simulink model "ex2"  (R2025b)
settings: Solver=VariableStepAuto  StartTime=0.0  StopTime=0.6  FixedStep=1e-4  RelTol=1e-4
values from neighbouring files (symbols this model uses):
  al = ap * 10    [sim3.m]
  Id_ref = psi_nominal_pu*psi_base/L_M    [sim3.m]
  Iq_ref = Te_nominal / ((3/2*K^2) * np * psi_nominal_pu*psi_base)    [sim3.m]
  ki = ac*(R_s+R_R+R_a)    [sim3.m]
  kip = ap*ap/psi_nominal    [sim3.m]
  kp = ac*L_sig    [sim3.m]
  kpp = 2*ap/psi_nominal    [sim3.m]
  L_sig = 0.0416    [sim3.m]
  R_a = ac*L_sig -(R_s+R_R)    [sim3.m]
  Te_nominal = Te_base * k    [sim3.m]
settings Model: Creator=Dimitris  LastModifiedBy=Dimitris

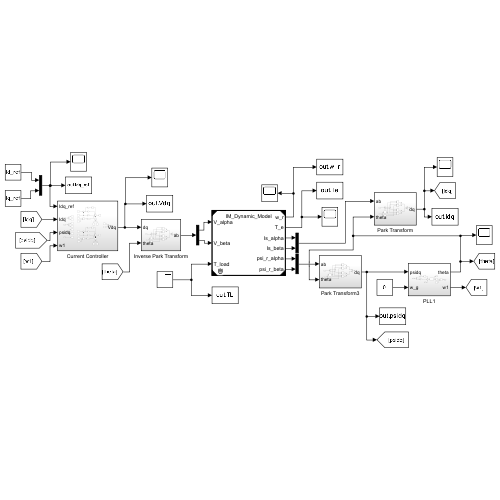
[thumbnail: Simulink's stored preview of the top-level diagram]
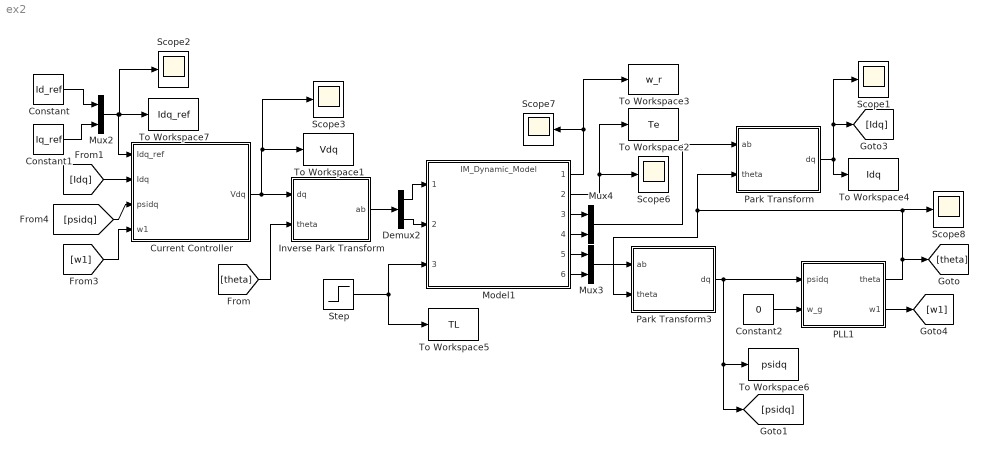
== system ex2 ==
  Constant : Constant  Value=Id_ref
  Constant1 : Constant  Value=Iq_ref
  Constant2 : Constant  Value=0
  Current Controller : Subsystem
  Demux2 : Demux  Outputs=2
  Inverse Park Transform : Subsystem
  Model1 : ModelReference  ModelNameDialog=IM_Dynamic_Model.slxp  ModelReferenceVersion=1.0  CopyOfModelProtected=on
  Mux2 : Mux  Inputs=2
  Mux3 : Mux  Inputs=2
  Mux4 : Mux  Inputs=2
  PLL1 : Subsystem
  Park Transform : Subsystem
  Park Transform3 : Subsystem
  Scope{1..3,6..8} (6 alike) : Scope
      Scope1 settings: ActiveDisplayYMinimum=-1.5675361173951203  ActiveDisplayYMaximum=7.0785524882099722
      Scope2 settings: ActiveDisplayYMinimum=0.8  ActiveDisplayYMaximum=2.8  DataLoggingVariableName=ScopeData2
      Scope3 settings: ActiveDisplayYMinimum=-366.50801253173779  ActiveDisplayYMaximum=2052.3481135758693  DataLoggingVariableName=ScopeData3
      Scope6 settings: ActiveDisplayYMinimum=-2.2517619671531257  ActiveDisplayYMaximum=20.265857704375257
      Scope7 settings: ActiveDisplayYMinimum=-65.744428661718672  ActiveDisplayYMaximum=591.69985795532909  DataLoggingVariableName=ScopeData6
      Scope8 settings: ActiveDisplayYMinimum=-0.78539816339744806  ActiveDisplayYMaximum=7.0685834705770345  DataLoggingVariableName=ScopeData7
  Step : Step  Time=0.3  After=Te_nominal*0.8  SampleTime=0
  To Workspace1 : ToWorkspace  VariableName=Vdq  SaveFormat=Timeseries  SampleTime=-1
  To Workspace2 : ToWorkspace  VariableName=Te  SaveFormat=Timeseries  SampleTime=-1
  To Workspace3 : ToWorkspace  VariableName=w_r  SaveFormat=Timeseries  SampleTime=-1
  To Workspace4 : ToWorkspace  VariableName=Idq  SaveFormat=Timeseries  SampleTime=-1
  To Workspace5 : ToWorkspace  VariableName=TL  SaveFormat=Timeseries  SampleTime=-1
  To Workspace6 : ToWorkspace  VariableName=psidq  SaveFormat=Timeseries  SampleTime=-1
  To Workspace7 : ToWorkspace  VariableName=Idq_ref  SaveFormat=Timeseries  SampleTime=-1
  wires:
  Current Controller/1(Vdq) -> Scope3/1, To Workspace1/1, Inverse Park Transform/1(dq)
  [Idq] -> Current Controller/2(Idq)
  Mux2/1 -> Scope2/1, To Workspace7/1, Current Controller/1(Idq_ref)
  Constant1/1 -> Mux2/2
  Constant/1 -> Mux2/1
  Inverse Park Transform/1(ab) -> Demux2/1
  PLL1/1(theta) -> Scope8/1, Park Transform3/2(theta), Park Transform/2(theta), [theta]
  Constant2/1 -> PLL1/2(w_g)
  Model1/4 -> Mux4/2
  Mux4/1 -> Park Transform/1(ab)
  Demux2/1 -> Model1/1
  Park Transform/1(dq) -> To Workspace4/1, [Idq], Scope1/1
  Step/1 -> To Workspace5/1, Model1/3
  Mux3/1 -> Park Transform3/1(ab)
  Demux2/2 -> Model1/2
  Model1/3 -> Mux4/1
  Model1/2 -> To Workspace2/1, Scope6/1
  Model1/6 -> Mux3/2
  Park Transform3/1(dq) -> [psidq], To Workspace6/1, PLL1/1(psidq)
  Model1/1 -> To Workspace3/1, Scope7/1
  Model1/5 -> Mux3/1
  [theta] -> Inverse Park Transform/2(theta)
  [psidq] -> Current Controller/3(psidq)
  [w1] -> Current Controller/4(w1)
  PLL1/2(w1) -> [w1]

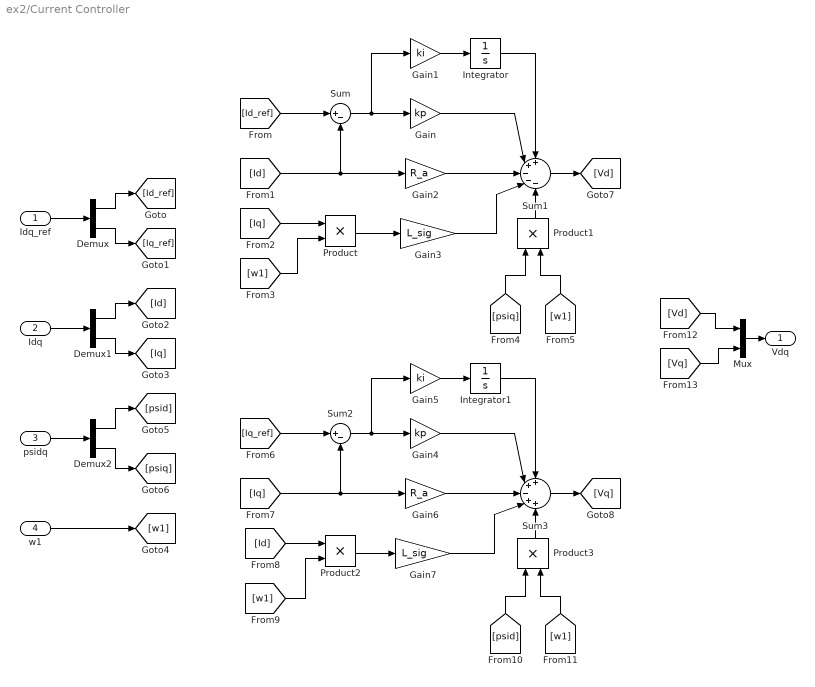
== system ex2/Current Controller ==
  Idq_ref : Inport
  Idq : Inport  Port=2
  psidq : Inport  Port=3
  w1 : Inport  Port=4
  Demux : Demux  Outputs=2
  Demux1 : Demux  Outputs=2
  Demux2 : Demux  Outputs=2
  Gain : Gain  Gain=kp
  Gain1 : Gain  Gain=ki
  Gain2 : Gain  Gain=R_a
  Gain3 : Gain  Gain=L_sig
  Gain4 : Gain  Gain=kp
  Gain5 : Gain  Gain=ki
  Gain6 : Gain  Gain=R_a
  Gain7 : Gain  Gain=L_sig
  Integrator : Integrator
  Integrator1 : Integrator
  Mux : Mux  Inputs=2
  Product{,1..3} (4 alike) : Product
  Sum : Sum  Inputs=|+-
  Sum1 : Sum  Inputs=++---
  Sum2 : Sum  Inputs=|+-
  Sum3 : Sum  Inputs=++-++
  Vdq : Outport
  wires:
  Idq_ref/1 -> Demux/1
  Mux/1 -> Vdq/1
  Idq/1 -> Demux1/1
  Demux/1 -> [Id_ref]
  Demux/2 -> [Iq_ref]
  Demux1/1 -> [Id]
  Demux1/2 -> [Iq]
  [Id_ref] -> Sum/1
  [Id] -> Sum/2, Gain2/1
  Sum/1 -> Gain1/1, Gain/1
  Gain1/1 -> Integrator/1
  Integrator/1 -> Sum1/1
  Gain/1 -> Sum1/2
  Gain2/1 -> Sum1/3
  Gain3/1 -> Sum1/4
  Product/1 -> Gain3/1
  w1/1 -> [w1]
  [Iq] -> Product/1
  [w1] -> Product/2
  psidq/1 -> Demux2/1
  Demux2/1 -> [psid]
  Demux2/2 -> [psiq]
  [psiq] -> Product1/1
  [w1] -> Product1/2
  Product1/1 -> Sum1/5
  Product3/1 -> Sum3/5
  [w1] -> Product3/2
  [psid] -> Product3/1
  Product2/1 -> Gain7/1
  [Id] -> Product2/1
  Integrator1/1 -> Sum3/1
  Gain6/1 -> Sum3/3
  Gain5/1 -> Integrator1/1
  Gain7/1 -> Sum3/4
  Sum2/1 -> Gain5/1, Gain4/1
  [Iq_ref] -> Sum2/1
  [w1] -> Product2/2
  [Iq] -> Sum2/2, Gain6/1
  Gain4/1 -> Sum3/2
  Sum1/1 -> [Vd]
  [Vd] -> Mux/1
  Sum3/1 -> [Vq]
  [Vq] -> Mux/2

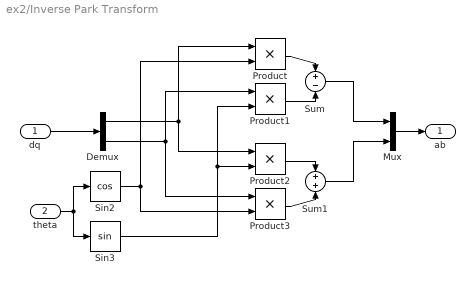
== system ex2/Inverse Park Transform ==
  dq : Inport
  theta : Inport  Port=2
  Demux : Demux  Outputs=2
  Mux : Mux  Inputs=2
  Product{,1..3} (4 alike) : Product
  Sin2 : Trigonometry  Operator=cos
  Sin3 : Trigonometry
  Sum : Sum  Inputs=+-
  Sum1 : Sum
  ab : Outport
  wires:
  Sum1/1 -> Mux/2
  Sin3/1 -> Product2/2, Product1/2
  Product1/1 -> Sum/2
  Demux/1 -> Product2/1, Product/1
  Mux/1 -> ab/1
  dq/1 -> Demux/1
  Sin2/1 -> Product/2, Product3/2
  Demux/2 -> Product1/1, Product3/1
  theta/1 -> Sin3/1, Sin2/1
  Sum/1 -> Mux/1
  Product/1 -> Sum/1
  Product3/1 -> Sum1/2
  Product2/1 -> Sum1/1

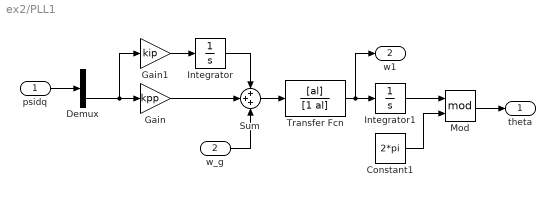
== system ex2/PLL1 ==
  psidq : Inport
  w_g : Inport  Port=2
  Constant1 : Constant  Value=2*pi
  Demux : Demux  Outputs=2
  Gain : Gain  Gain=kpp
  Gain1 : Gain  Gain=kip
  Integrator : Integrator
  Integrator1 : Integrator
  Mod : Math  Operator=mod
  Sum : Sum  Inputs=+++
  Transfer Fcn : TransferFcn  Numerator=[al]  Denominator=[1 al]
  theta : Outport
  w1 : Outport  Port=2
  wires:
  Gain1/1 -> Integrator/1
  Gain/1 -> Sum/2
  Sum/1 -> Transfer Fcn/1
  Transfer Fcn/1 -> w1/1, Integrator1/1
  Constant1/1 -> Mod/2
  Integrator1/1 -> Mod/1
  Mod/1 -> theta/1
  Demux/2 -> Gain1/1, Gain/1
  psidq/1 -> Demux/1
  Integrator/1 -> Sum/1
  w_g/1 -> Sum/3

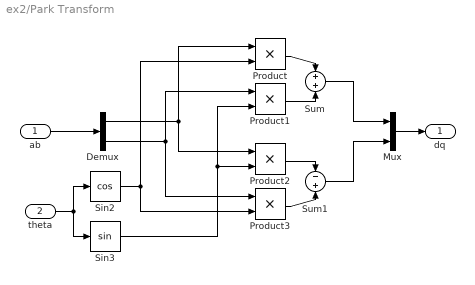
== system ex2/Park Transform ==
  ab : Inport
  theta : Inport  Port=2
  Demux : Demux  Outputs=2
  Mux : Mux  Inputs=2
  Product{,1..3} (4 alike) : Product
  Sin2 : Trigonometry  Operator=cos
  Sin3 : Trigonometry
  Sum : Sum
  Sum1 : Sum  Inputs=-+
  dq : Outport
  wires:
  Sin3/1 -> Product1/2, Product2/2
  Sin2/1 -> Product/2, Product3/2
  theta/1 -> Sin3/1, Sin2/1
  Demux/2 -> Product1/1, Product3/1
  Sum1/1 -> Mux/2
  Sum/1 -> Mux/1
  Demux/1 -> Product2/1, Product/1
  Product2/1 -> Sum1/1
  Product3/1 -> Sum1/2
  Product1/1 -> Sum/2
  Product/1 -> Sum/1
  Mux/1 -> dq/1
  ab/1 -> Demux/1

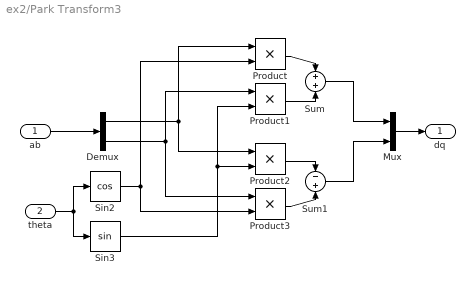
== system ex2/Park Transform3 ==
  ab : Inport
  theta : Inport  Port=2
  Demux : Demux  Outputs=2
  Mux : Mux  Inputs=2
  Product{,1..3} (4 alike) : Product
  Sin2 : Trigonometry  Operator=cos
  Sin3 : Trigonometry
  Sum : Sum
  Sum1 : Sum  Inputs=-+
  dq : Outport
  wires:
  Sin3/1 -> Product1/2, Product2/2
  Sin2/1 -> Product/2, Product3/2
  theta/1 -> Sin3/1, Sin2/1
  Demux/2 -> Product1/1, Product3/1
  Sum1/1 -> Mux/2
  Sum/1 -> Mux/1
  Demux/1 -> Product2/1, Product/1
  Product2/1 -> Sum1/1
  Product3/1 -> Sum1/2
  Product1/1 -> Sum/2
  Product/1 -> Sum/1
  Mux/1 -> dq/1
  ab/1 -> Demux/1
